simulink model "UAM_Hexa_PD_Obs_Disc"  (R2026a)
settings: Solver=ode4  StopTime=40  FixedStep=st
values from neighbouring files (symbols this model uses):
  ArmConstants = struct('l1_dim', l1_dim,                        'l2_dim', l2_dim,                        'Hexa_to_joint_L', L,                        'Mass1', ml1,                        'Mass2', ml2,                        'Inertia1', Hl1,                        'Inertia2', Hl2,                        'MC1', c1,                        'MC2', c2,                        'Servos', Servos)    [init_model.m]    (also in init_var.m)
  HexaConstants = struct('Mass', mb,                         'Inertia', J ,                         'allo', allo,                          'invallo', invallo,                         'kT', kT)    [init_model.m]    (also in init_var.m)
  Observer = struct('E1', E1 ,     'E2', E2 ,     'E3', E3 ,     'E4', E4 ,     'MU1', MU1 ,     'MU2', MU2 ,     'MU3', MU3 ,     'alpha', alpha ,     'beta', beta)    [init_model.m]    (also in init_var.m)
  PID = InitController()    [init_model.m]    (also in init_var.m)
  st = 0.01    [init_model.m]    (also in init_var.m; px4HostTarget_TCPIP_Read.m = matlab.system.SampleTimeSpecification('Type', 'Discrete',   )
undefined symbols (not defined in the file or in its folder): DiscIntNeverNeededParam
settings Model: Creator=Carlos Fabian  LastModifiedBy=Carlos Fabian
settings ExplorerConfigSet: InternalSimMechanicsExplorerSettings=|
  | <ExplorerConfiguration>
  | 
  |   <canonicalview>default</canonicalview>
  | 
  |   <TilePanel>
  |     <TileInfo>
  |       <Tiles Columns="1" Count="1" Height="513" Rows="1" Width="774">
  |         <Row Weight="1"/>
  |         <Column Weight="1"/>
  |         <Tile Height="1" Width="1" X="0" Y="0"/>
  |       </Tiles>
  |     </TileInfo>
  |     <SceneInfo>
  |       <SceneViewer>
  |         <IsThisViewStd>
  |           <IsStandardView>off</IsStandardView>
  |           <StandardViewName>Front</StandardViewName>
  |         </IsThisViewStd>
  |         <BGColor>
  |           <R>1</R>
  |           <G>1</G>
  |           <B>1</B>
  |           <A>1</A>
  |         </BGColor>
  |         <Camera>
  |           <DoPerspective>off</DoPerspective>
  |           <Position>
  |             <X>16.201091586104312</X>
  |             <Y>-16.65504514146788</Y>
  |             <Z>17.087073385082522</Z>
  |           </Position>
  |           <Center>
  |             <X>-0.25720946651222221</X>
  |             <Y>-0.19674408885134653</Y>
  |             <Z>0.62877233246599318</Z>
  |           </Center>
  |           <Up>
  |             <X>-0.40824829046386302</X>
  |             <Y>0.40824829046386302</Y>
  |             <Z>0.81649658092772615</Z>
  |           </Up>
  |           <XLim>2.5491252053936631</XLim>
  |           <YLim>2.5491252053936631</YLim>
  |           <ViewLimDist>0.01</ViewLimDist>
  |         </Camera>
  |       </SceneViewer>
  |     </SceneInfo>
  |   </TilePanel>
  | 
  |   <MechEditorPanel>
  |     <GfxPanelCameraMap/>
  |     <Cameras/>
  |     <VideoCreator>
  |       <IncludeTiles>All</IncludeTiles>
  |       <IncludeTime>on</IncludeTime>
  |       <IncludeWorldFrame>off</IncludeWorldFrame>
  |       <PlaybackSpeedRatio>8</PlaybackSpeedRatio>
  |       <FrameRate>24</FrameRate>
  |       <FrameSize>auto</FrameSize>
  |       <VideoFormat>MotionJPEGAVI</VideoFormat>
  |     </VideoCreator>
  |   </MechEditorPanel>
  | 
  |   <PlaybackSettings>
  |     <PlaybackSpeedFactor>16</PlaybackSpeedFactor>
  |   </PlaybackSettings>
  | 
  | </ExplorerConfiguration>

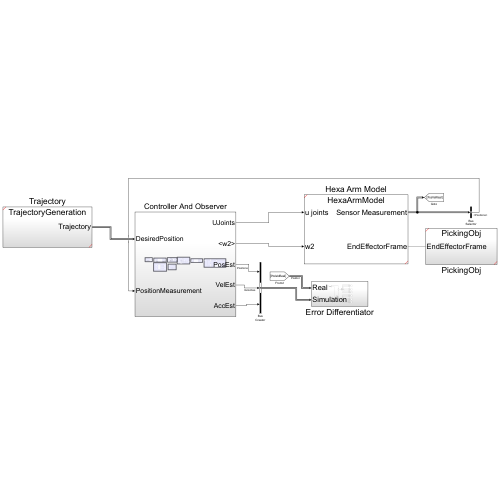
[thumbnail: Simulink's stored preview of the top-level diagram]
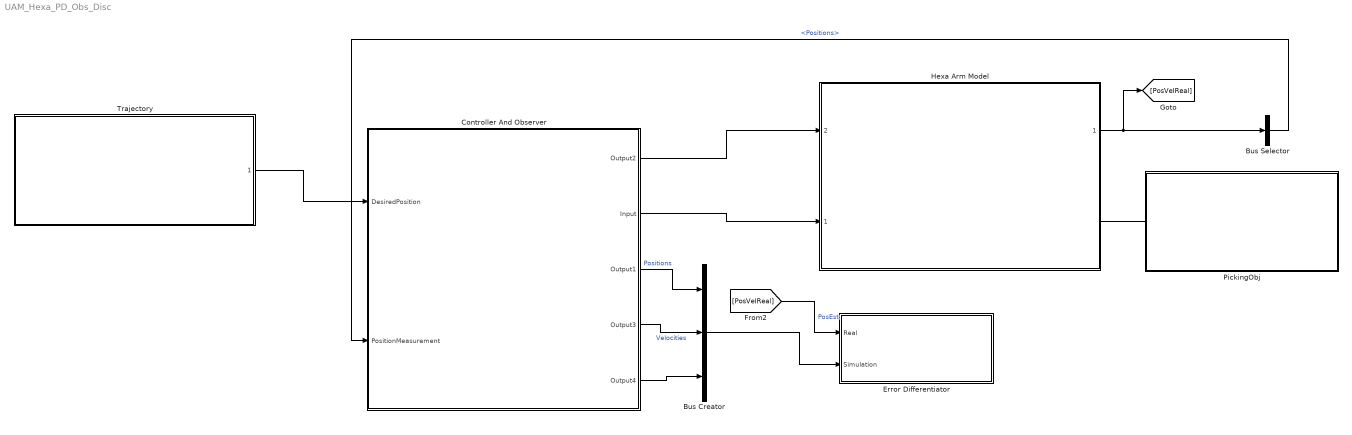
== system UAM_Hexa_PD_Obs_Disc ==
  Bus Creator : BusCreator  Inputs=3
  Bus Selector : BusSelector  OutputSignals=Positions
  Controller And Observer : Subsystem
  Error Differentiator : Subsystem
  Hexa Arm Model : Subsystem  ReferencedSubsystem=HexaArmModel
      settings: PortSchema="{\"entries\":[{\"content\":{\"sides\":[{\"content\":{\"connectorIds\":[\"In2\",\"In1\"]},\"type\":\"ConnectorPlacement.EquallySpacedRectSide\",\"uuid\":\"8c321911-c61a-4c60-b031-eeaf4c8b5083\"},{\"content\":{\"connectorIds\":[\"Out1\",\"RConn1\"],\"side\":\"RIGHT\"},\"type\":\"ConnectorPlacement.EquallySpacedRectSide\",\"uuid\":\"3ad1588f-e2f8-4666-8b86-318f5207193d\"},{\"content\":{\"side\":\"TOP\"},\"type\":\"ConnectorPlacement.EquallySpacedRectSide\",\"uuid\":\"710cc49c-59c4-4f69-a558-4588d1d119c0\"}]},\"type\":\"ConnectorPlacement.EquallySpacedConnector\",\"uuid\":\"3e8cca1f-f7f1-4f31-9eba-ef93ff8e81e8\"}],\"packageUris\":[\"http://schema.mathworks.com/mf0/Connector/R2020b\"],\"version\":\"1.0\"}"
  PickingObj : Subsystem  ReferencedSubsystem=PickingObj
  Trajectory : Subsystem  ReferencedSubsystem=TrajectoryGeneration
  wires:
  Controller And Observer/2(Input) -> Hexa Arm Model/1
  Trajectory/1 -> Controller And Observer/1(DesiredPosition)
  Hexa Arm Model/1 -> [PosVelReal], Bus Selector/1
  Controller And Observer/1(Output2) -> Hexa Arm Model/2
  Bus Selector/1 -> Controller And Observer/2(PositionMeasurement)  "<Positions>"
  [PosVelReal] -> Error Differentiator/1(Real)  "PosEst"
  Controller And Observer/4(Output3) -> Bus Creator/2  "Velocities"
  Controller And Observer/3(Output1) -> Bus Creator/1  "Positions"
  Bus Creator/1 -> Error Differentiator/2(Simulation)
  Controller And Observer/5(Output4) -> Bus Creator/3
  connections:
  Hexa Arm Model/RConn1 -- PickingObj/LConn1

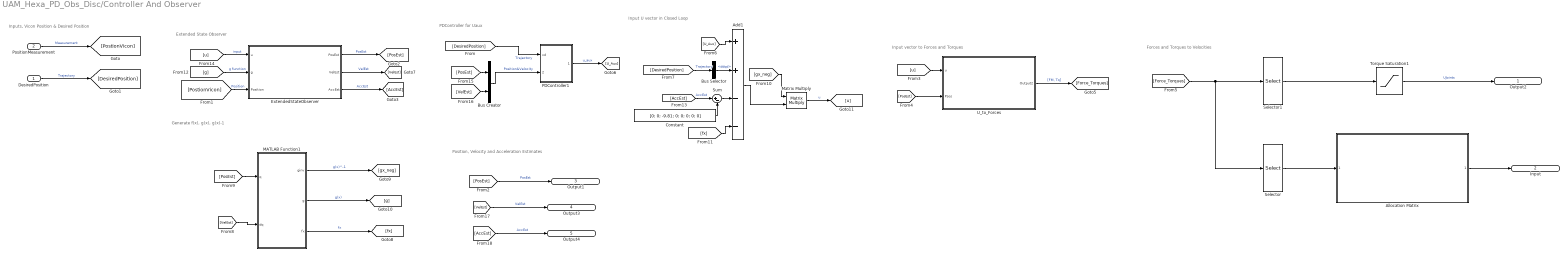
== system UAM_Hexa_PD_Obs_Disc/Controller And Observer ==
  note: Position, Velocity and Acceleration Estimates
  note: Input vector to Forces and Torques
  note: Forces and Torques to Velocities
  note: Extended State Observer
  note: Input U vector in Closed Loop
  note: Generate f(x), g(x), g(x)-1
  note: PDController for Uaux
  note: Inputs, Vicon Position & Desired Position
  DesiredPosition : Inport
  PositionMeasurement : Inport  Port=2
  Add1 : Sum  Inputs=++--
  Allocation Matrix : Subsystem  ReferencedSubsystem=FromFMtoOmega2
  Bus Creator : BusCreator  Inputs=2
  Bus Selector : BusSelector  OutputSignals=ddqd
  Constant : Constant  Value=[0; 0; -9.81; 0; 0; 0; 0; 0]
  ExtendedStateObserver : Subsystem
  MATLAB Function1 : MATLAB Function  TreatAsAtomicUnit=on
  Matrix Multiply : Product  Multiplication=Matrix(*)
  PDController1 : Subsystem
  Selector : Selector  InputPortWidth=8  IndexOptions=Index vector (dialog)  Indices=1:6  OutputSizes=1
  Selector1 : Selector  InputPortWidth=8  IndexOptions=Index vector (dialog)  Indices=7:8  OutputSizes=1
  Sum : Sum  Inputs=|+-
  Torque Saturation1 : Saturate  UpperLimit=ArmConstants.Servos.T1max  LowerLimit=-ArmConstants.Servos.T1max
  U_to_Forces : Subsystem
  Output2 : Outport
  Input : Outport  Port=2
  Output1 : Outport  Port=3
  Output3 : Outport  Port=4
  Output4 : Outport  Port=5
  wires:
  [PostionVicon] -> ExtendedStateObserver/3(Position)  "Position"
  [DesiredPosition] -> PDController1/1(xd)  "Trajectory"
  U_to_Forces/1(Output2) -> [Force_Torques]  "[FM, Tq]"
  ExtendedStateObserver/1(PosEst) -> [PosEst]  "PosEst"
  PositionMeasurement/1 -> [PostionVicon]  "Measurement"
  DesiredPosition/1 -> [DesiredPosition]  "Trajectory"
  Bus Creator/1 -> PDController1/2(q_hat1)  "Position&Velocity"
  ExtendedStateObserver/3(AccEst) -> [AccEst]  "AccEst"
  ExtendedStateObserver/2(VelEst) -> [VelEst]  "VelEst"
  [PosEst] -> U_to_Forces/2(Psos)
  Selector1/1 -> Torque Saturation1/1
  [Force_Torques] -> Selector/1, Selector1/1
  Selector/1 -> Allocation Matrix/1
  Torque Saturation1/1 -> Output2/1  "UJoints"
  Allocation Matrix/1 -> Input/1
  PDController1/1(Output) -> [U_Aux]  "u_aux"
  MATLAB Function1/1(ginv) -> [gx_neg]  "g(x)^-1"
  MATLAB Function1/3(fx) -> [fx]  "fx"
  [VelEst] -> MATLAB Function1/2(dq)
  [PosEst] -> MATLAB Function1/1(q)
  [fx] -> Add1/4
  Add1/1 -> Matrix Multiply/2
  Matrix Multiply/1 -> [u]  "u"
  [gx_neg] -> Matrix Multiply/1
  [U_Aux] -> Add1/1
  [DesiredPosition] -> Bus Selector/1  "Trajectory"
  Bus Selector/1 -> Add1/2  "<ddqd>"
  [AccEst] -> Sum/1  "AccEst"
  MATLAB Function1/2(g) -> [g]  "g(x)"
  [g] -> ExtendedStateObserver/2(g)  "g function"
  [u] -> ExtendedStateObserver/1(u)  "input"
  [PosEst] -> Bus Creator/1
  [VelEst] -> Bus Creator/2
  [u] -> U_to_Forces/1(u)
  [PosEst] -> Output1/1  "PosEst"
  [VelEst] -> Output3/1  "VelEst"
  [AccEst] -> Output4/1  "AccEst"
  Sum/1 -> Add1/3
  Constant/1 -> Sum/2

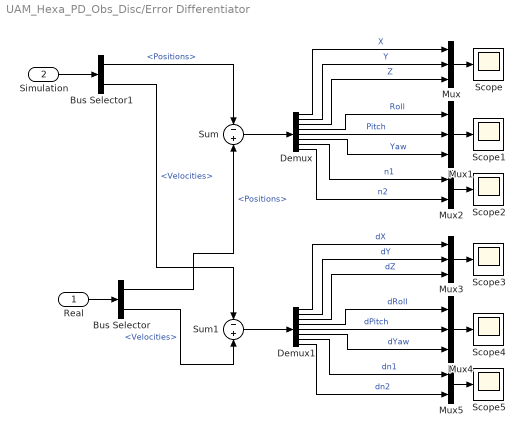
== system UAM_Hexa_PD_Obs_Disc/Error Differentiator ==
  Real : Inport
  Simulation : Inport  Port=2
  Bus Selector : BusSelector  OutputSignals=Positions,Velocities
  Bus Selector1 : BusSelector  OutputSignals=Positions,Velocities
  Demux : Demux  Outputs=8
  Demux1 : Demux  Outputs=8
  Mux{,1,3..4} (4 alike) : Mux  Inputs=3
  Mux2 : Mux  Inputs=2
  Mux5 : Mux  Inputs=2
  Scope{,1..5} (6 alike) : Scope
      Scope settings: ActiveDisplayYMinimum=-0.12805242657923774  ActiveDisplayYMaximum=0.1215294954009426
      Scope1 settings: ActiveDisplayYMinimum=-0.0054009288599574049  ActiveDisplayYMaximum=0.0052845116621625422  DataLoggingVariableName=ScopeData4
      Scope2 settings: ActiveDisplayYMinimum=-0.13481735348450222  ActiveDisplayYMaximum=0.11770569677593748  DataLoggingVariableName=ScopeData5
      Scope3 settings: ActiveDisplayYMinimum=-0.04776683780805524  ActiveDisplayYMaximum=0.068912520834715912  DataLoggingVariableName=ScopeData6
      Scope4 settings: ActiveDisplayYMinimum=-0.051890288196585518  ActiveDisplayYMaximum=0.072205334726900258  DataLoggingVariableName=ScopeData7
      Scope5 settings: ActiveDisplayYMinimum=-4.0019143526268195  ActiveDisplayYMaximum=18.067364456962562  DataLoggingVariableName=ScopeData8
  Sum : Sum  Inputs=-+
  Sum1 : Sum  Inputs=-+
  wires:
  Mux2/1 -> Scope2/1
  Sum/1 -> Demux/1
  Mux1/1 -> Scope1/1
  Bus Selector1/1 -> Sum/1  "<Positions>"
  Demux/8 -> Mux2/2  "n2"
  Bus Selector/2 -> Sum1/2  "<Velocities>"
  Demux/7 -> Mux2/1  "n1"
  Mux/1 -> Scope/1
  Demux/1 -> Mux/1  "X"
  Demux/4 -> Mux1/1  "Roll"
  Demux/6 -> Mux1/3  "Yaw"
  Demux/5 -> Mux1/2  "Pitch"
  Demux/3 -> Mux/3  "Z"
  Bus Selector/1 -> Sum/2  "<Positions>"
  Demux/2 -> Mux/2  "Y"
  Bus Selector1/2 -> Sum1/1  "<Velocities>"
  Simulation/1 -> Bus Selector1/1
  Real/1 -> Bus Selector/1
  Demux1/8 -> Mux5/2  "dn2"
  Mux4/1 -> Scope4/1
  Sum1/1 -> Demux1/1
  Mux5/1 -> Scope5/1
  Demux1/4 -> Mux4/1  "dRoll"
  Demux1/6 -> Mux4/3  "dYaw"
  Demux1/2 -> Mux3/2  "dY"
  Demux1/1 -> Mux3/1  "dX"
  Mux3/1 -> Scope3/1
  Demux1/5 -> Mux4/2  "dPitch"
  Demux1/7 -> Mux5/1  "dn1"
  Demux1/3 -> Mux3/3  "dZ"

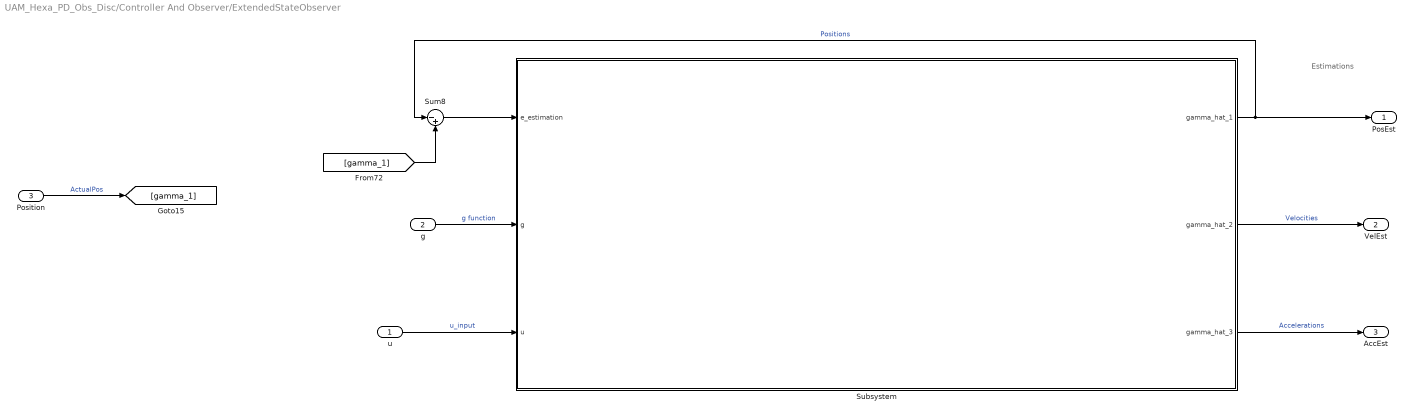
== system UAM_Hexa_PD_Obs_Disc/Controller And Observer/ExtendedStateObserver ==
  note: Estimations
  u : Inport
  g : Inport  Port=2
  Position : Inport  Port=3
  Subsystem : Subsystem
  Sum8 : Sum  Inputs=|-+
  PosEst : Outport
  VelEst : Outport  Port=2
  AccEst : Outport  Port=3
  wires:
  Subsystem/1(gamma_hat_1) -> PosEst/1, Sum8/1  "Positions"
  [gamma_1] -> Sum8/2
  u/1 -> Subsystem/3(u)  "u_input"
  Position/1 -> [gamma_1]  "ActualPos"
  g/1 -> Subsystem/2(g)  "g function"
  Subsystem/3(gamma_hat_3) -> AccEst/1  "Accelerations"
  Subsystem/2(gamma_hat_2) -> VelEst/1  "Velocities"
  Sum8/1 -> Subsystem/1(e_estimation)

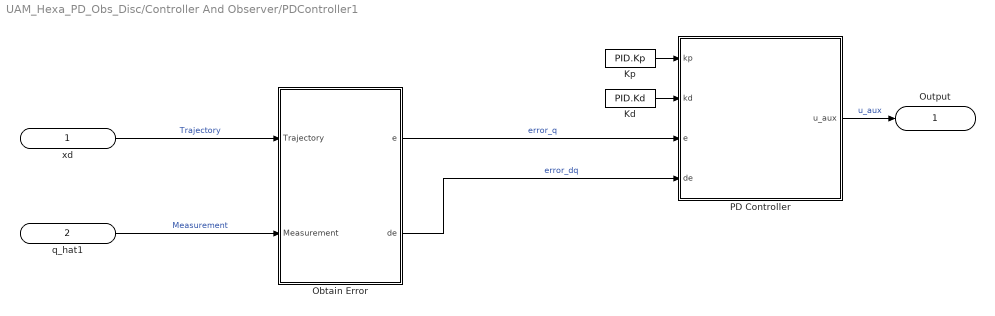
== system UAM_Hexa_PD_Obs_Disc/Controller And Observer/PDController1 ==
  xd : Inport
  q_hat1 : Inport  Port=2
  Kd : Constant  Value=PID.Kd
  Kp : Constant  Value=PID.Kp
  Obtain Error : Subsystem
  PD Controller : MATLAB Function  TreatAsAtomicUnit=on
  Output : Outport
  wires:
  xd/1 -> Obtain Error/1(Trajectory)  "Trajectory"
  q_hat1/1 -> Obtain Error/2(Measurement)  "Measurement"
  Obtain Error/1(e) -> PD Controller/3(e)  "error_q"
  Obtain Error/2(de) -> PD Controller/4(de)  "error_dq"
  Kp/1 -> PD Controller/1(kp)
  Kd/1 -> PD Controller/2(kd)
  PD Controller/1(u_aux) -> Output/1  "u_aux"

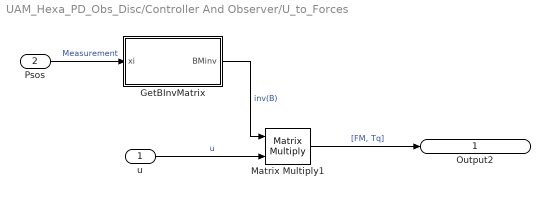
== system UAM_Hexa_PD_Obs_Disc/Controller And Observer/U_to_Forces ==
  u : Inport
  Psos : Inport  Port=2
  GetBInvMatrix : MATLAB Function  TreatAsAtomicUnit=on
  Matrix Multiply1 : Product  Multiplication=Matrix(*)
  Output2 : Outport
  wires:
  Psos/1 -> GetBInvMatrix/1(xi)  "Measurement"
  u/1 -> Matrix Multiply1/2  "u"
  Matrix Multiply1/1 -> Output2/1  "[FM, Tq]"
  GetBInvMatrix/1(BMinv) -> Matrix Multiply1/1  "inv(B)"

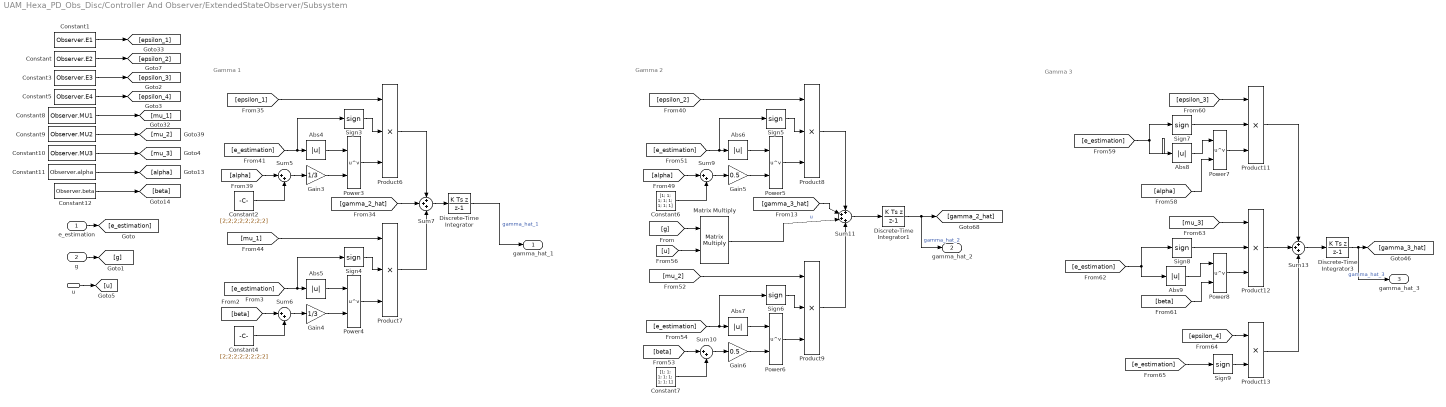
== system UAM_Hexa_PD_Obs_Disc/Controller And Observer/ExtendedStateObserver/Subsystem ==
  note: Gamma 3
  note: Gamma 2
  note: Gamma 1
  e_estimation : Inport
  g : Inport  Port=2
  u : Inport  Port=3
  Abs{4..9} (6 alike) : Abs  SaturateOnIntegerOverflow=off
  Constant : Constant  Value=Observer.E2
  Constant1 : Constant  Value=Observer.E1
  Constant10 : Constant  Value=Observer.MU3
  Constant11 : Constant  Value=Observer.alpha
  Constant12 : Constant  Value=Observer.beta
  Constant2 : Constant  Value=[2;2;2;2;2;2;2;2]
  Constant3 : Constant  Value=Observer.E3
  Constant4 : Constant  Value=[2;2;2;2;2;2;2;2]
  Constant5 : Constant  Value=Observer.E4
  Constant6 : Constant  Value=[1; 1; 1; 1; 1; 1; 1; 1]
  Constant7 : Constant  Value=[1; 1; 1; 1; 1; 1; 1; 1]
  Constant8 : Constant  Value=Observer.MU1
  Constant9 : Constant  Value=Observer.MU2
  Discrete-Time Integrator : DiscreteIntegrator  IntegratorMethod=Integration: Backward Euler  InitialCondition=[0; 0; 0.24; 0; 0; 0; 0; 0]  SampleTime=st  ICPrevOutput=DiscIntNeverNeededParam  ICPrevScaledInput=DiscIntNeverNeededParam
  Discrete-Time Integrator1 : DiscreteIntegrator  IntegratorMethod=Integration: Backward Euler  InitialCondition=zeros(8,1)  SampleTime=st  ICPrevOutput=DiscIntNeverNeededParam  ICPrevScaledInput=DiscIntNeverNeededParam
  Discrete-Time Integrator3 : DiscreteIntegrator  IntegratorMethod=Integration: Backward Euler  InitialCondition=[0; 0; -9.81; 0; 0; 0; 0; 0]  SampleTime=st  ICPrevOutput=DiscIntNeverNeededParam  ICPrevScaledInput=DiscIntNeverNeededParam
  Gain3 : Gain  Gain=1/3
  Gain4 : Gain  Gain=1/3
  Gain5 : Gain  Gain=0.5
  Gain6 : Gain  Gain=0.5
  Matrix Multiply : Product  Multiplication=Matrix(*)
  Power{3..8} (6 alike) : Math  Operator=pow
  Product{6..9,11..12} (6 alike) : Product  Inputs=3
  Product13 : Product
  Sign{3..9} (7 alike) : Signum
  Sum{5..6,9..10} (4 alike) : Sum  Inputs=|++
  Sum11 : Sum  Inputs=++++
  Sum13 : Sum  Inputs=+++
  Sum7 : Sum  Inputs=+++
  gamma_hat_1 : Outport
  gamma_hat_2 : Outport  Port=2
  gamma_hat_3 : Outport  Port=3
  wires:
  Sum9/1 -> Gain5/1
  Sign6/1 -> Product9/2
  [e_estimation] -> Sign9/1
  [e_estimation] -> Sign3/1, Abs4/1
  Abs6/1 -> Power5/1
  [u] -> Matrix Multiply/2
  Power8/1 -> Product12/3
  [g] -> Matrix Multiply/1
  [alpha] -> Sum9/1
  Constant6/1 -> Sum9/2
  Constant2/1 -> Sum5/2
  Abs7/1 -> Power6/1
  Matrix Multiply/1 -> Sum11/3  "u"
  [beta] -> Power8/2
  [mu_3] -> Product12/1
  [epsilon_3] -> Product11/1
  Constant9/1 -> [mu_2]
  [mu_1] -> Product7/1
  Sum13/1 -> Discrete-Time Integrator3/1
  Product11/1 -> Sum13/1
  [e_estimation] -> Sign5/1, Abs6/1
  Product9/1 -> Sum11/4
  [e_estimation] -> Abs8/1, Sign7/1
  Constant/1 -> [epsilon_2]
  Sign5/1 -> Product8/2
  [beta] -> Sum6/1
  Constant5/1 -> [epsilon_4]
  Sum11/1 -> Discrete-Time Integrator1/1
  [gamma_3_hat] -> Sum11/2
  Abs5/1 -> Power4/1
  Sum6/1 -> Gain4/1
  Power5/1 -> Product8/3
  Product13/1 -> Sum13/3
  [gamma_2_hat] -> Sum7/2
  [e_estimation] -> Sign6/1, Abs7/1
  Sign7/1 -> Product11/2
  Sum10/1 -> Gain6/1
  Discrete-Time Integrator1/1 -> gamma_hat_2/1, [gamma_2_hat]  "gamma_hat_2"
  [alpha] -> Power7/2
  Discrete-Time Integrator3/1 -> gamma_hat_3/1, [gamma_3_hat]  "gamma_hat_3"
  Sign9/1 -> Product13/2
  Sign4/1 -> Product7/2
  Gain4/1 -> Power4/2
  Constant11/1 -> [alpha]
  Sum7/1 -> Discrete-Time Integrator/1
  Discrete-Time Integrator/1 -> gamma_hat_1/1  "gamma_hat_1"
  Gain5/1 -> Power5/2
  Constant12/1 -> [beta]
  [alpha] -> Sum5/1
  Sum5/1 -> Gain3/1
  Constant7/1 -> Sum10/2
  Abs8/1 -> Power7/1
  Sign8/1 -> Product12/2
  Product12/1 -> Sum13/2
  Abs9/1 -> Power8/1
  [epsilon_2] -> Product8/1
  Power6/1 -> Product9/3
  Constant3/1 -> [epsilon_3]
  Sign3/1 -> Product6/2
  Gain6/1 -> Power6/2
  Power4/1 -> Product7/3
  Constant8/1 -> [mu_1]
  Constant1/1 -> [epsilon_1]
  [epsilon_4] -> Product13/1
  [e_estimation] -> Sign4/1, Abs5/1
  [epsilon_1] -> Product6/1
  Abs4/1 -> Power3/1
  Product7/1 -> Sum7/3
  [beta] -> Sum10/1
  Constant4/1 -> Sum6/2
  Constant10/1 -> [mu_3]
  [e_estimation] -> Sign8/1, Abs9/1
  Power3/1 -> Product6/3
  Power7/1 -> Product11/3
  Gain3/1 -> Power3/2
  Product8/1 -> Sum11/1
  Product6/1 -> Sum7/1
  [mu_2] -> Product9/1
  e_estimation/1 -> [e_estimation]
  g/1 -> [g]
  u/1 -> [u]

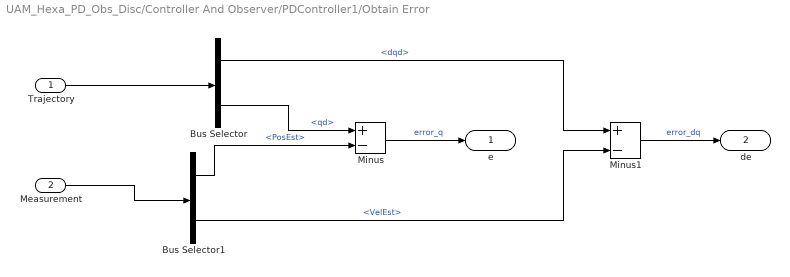
== system UAM_Hexa_PD_Obs_Disc/Controller And Observer/PDController1/Obtain Error ==
  Trajectory : Inport
  Measurement : Inport  Port=2
  Bus Selector : BusSelector  OutputSignals=dqd,qd
  Bus Selector1 : BusSelector  OutputSignals=PosEst,VelEst
  Minus : Sum  Inputs=+-
  Minus1 : Sum  Inputs=+-
  e : Outport
  de : Outport  Port=2
  wires:
  Bus Selector1/1 -> Minus/2  "<PosEst>"
  Bus Selector1/2 -> Minus1/2  "<VelEst>"
  Measurement/1 -> Bus Selector1/1
  Trajectory/1 -> Bus Selector/1
  Bus Selector/1 -> Minus1/1  "<dqd>"
  Bus Selector/2 -> Minus/1  "<qd>"
  Minus/1 -> e/1  "error_q"
  Minus1/1 -> de/1  "error_dq"

== matlab function UAM_Hexa_PD_Obs_Disc/Controller And Observer/PDController1/PD Controller ==
  data: kp input; kd input; u_aux output; e input; de input
function u_aux = pd_cont(kp, kd, e, de)


kp_m = [kp(1) 0       0     0     0       0     0     0;
        0     kp(2)   0     0     0       0     0     0;
        0     0       kp(3) 0     0       0     0     0;
        0     0       0     kp(4) 0       0     0     0;
        0     0       0     0     kp(5)   0     0     0;
        0     0       0     0     0       kp(6) 0     0;
        0     0       0     0     0       0     kp(7) 0;
        0     0       0     0     0       0     0     kp(8)];

kd_m = [kd(1) 0       0     0     0       0     0     0;
        0     kd(2)   0     0     0       0     0     0;
        0     0       kd(3) 0     0       0     0     0;
        0     0       0     kd(4) 0       0     0     0;
        0     0       0     0     kd(5)   0     0     0;
        0     0       0     0     0       kd(6) 0     0;
        0     0       0     0     0       0     kd(7) 0;
        0     0       0     0     0       0     0     kd(8)];


%v = ddP + kp_m * e + kd_m * de;
u_aux = kp_m * e + kd_m * de;
%v = ddP;

end

== matlab function UAM_Hexa_PD_Obs_Disc/Controller And Observer/MATLAB Function1 ==
  data: q input; dq input; HexaConstants parameter; ginv output; g output; fx output; ArmConstants parameter
function [ginv, g, fx] = Get_DCG_Hexa(q, dq, HexaConstants, ArmConstants)

DM = DMatrix(q, HexaConstants, ArmConstants);
CM = CMatrix(q, dq, HexaConstants, ArmConstants);
Gv = GVector(q, HexaConstants, ArmConstants);

g = inv(DM);
ginv = DM;

fx = DM\( -CM*dq - Gv );

end

== matlab function UAM_Hexa_PD_Obs_Disc/Controller And Observer/U_to_Forces/GetBInvMatrix ==
  data: xi input; BMinv output
function BMinv = GetBInvMatrix(xi)

% phi = xi(4);
% th  = xi(5);
% psi = xi(6);
% 
% BM1=[cos(phi)*cos(th),-cos(phi)*sin(psi)+cos(psi)*sin(phi)*sin(th), ...
%     sin(phi)*sin(psi)+cos(phi)*cos(psi)*sin(th),0,0,0;...
%     cos(th)*sin(psi), cos(phi)*cos(psi)+sin(phi)*sin(psi)*sin(th),...
%     -cos(psi)*sin(phi)+cos(phi)*sin(psi)*sin(phi),0,0,0;...
%     -sin(th),cos(th)*sin(psi),cos(phi)*cos(th),0,0,0;...
%     0,0,0,1,sin(phi)*tan(th),cos(phi)*tan(th);...
%     0,0,0,0,cos(phi),-sin(phi);0,0,0,0,sec(th)*sin(phi),cos(phi)*sec(th)];

BM1 = BMatrix(xi);

BM = blkdiag(BM1, eye(2,2));

BMinv = inv(BM);

end
